simulink model "baseline_source"  (R2025a)
settings: Solver=daessc  StartTime=0.0  StopTime=25  MaxStep=5e-6  RelTol=1e-3
model workspace (MAT data in the model file):
  FocDiscrTime = 8.33333333333e-05
  Is_max = 420
  Ld = 0.00031
  Lq = 0.000305
  PolePairs = 11
  Psi = 0.1024
  Rs = 0.02
  VDC = 440
  compensate_dt = 0
  compensate_pwm = 0
  deltaLd = 0
  deltaLq = 0
  deltaPsi = 0
  deltaRs = 0
  mFW = 0.95
  mMaxCurrent = 0.99
  mMaxPWM = 0.99
  piBandwidth = 6000
libraries: fl_lib x18, nesl_utility x15, eeGeneralControl x9, mcbeeMathTransformLib x7, simulink x7, slpidlib x5, spsMeanLib x4, ee_lib x1, simulink_extras x1
(part 2 of 2)

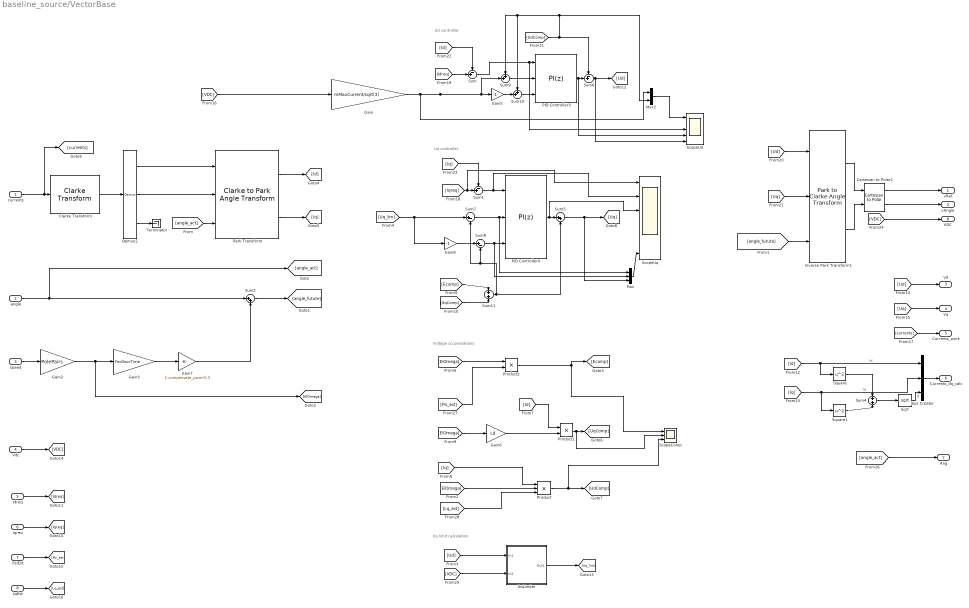
== system baseline_source/VectorBase ==
  note: Uq limit calculation
  note: Voltage co,pensations
  note: Ud controller
  note: Uq controller
  currents : Inport
  angle : Inport  Port=2
  speed : Inport  Port=3
  Vdc : Inport  Port=4
  Idreq : Inport  Port=5
  Iqreq : Inport  Port=6
  PsiEst : Inport  Port=7
  LqEst : Inport  Port=8
  Bus Creator : BusCreator  Inputs=3
  Cartesian to Polar1 : simulink_extras/Transformations/Cartesian to Polar
  Clarke Transform : mcbeeMathTransformLib/Clarke Transform  VariantControl=Variant2  PowerInvariant=off  UseWithEmbedded=on  PhaseInput=Three inputs
      settings: LibrarySourceBlock=mcbcontrolslib/Clarke Transform
  Demux2 : Demux  Outputs=3
  Gain : Gain  Gain=mMaxCurrent/sqrt(3)
  Gain2 : Gain  Gain=PolePairs
  Gain3 : Gain  Gain=FocDiscrTime
  Gain5 : Gain  Gain=-1
  Gain6 : Gain  Gain=Ld
  Gain7 : Gain  Gain=1-compensate_pwm*0.5
  Gain8 : Gain  Gain=-1
  Inverse Park Transform1 : mcbeeMathTransformLib/Park to Clarke Angle Transform  AxisAlignment=D-axis  UseWithEmbedded=on  PhaseInput=Two inputs  ThetaInput=Electrical position  AngleInput=Radians  N_points=1024
      settings: LibrarySourceBlock=mcbcontrolslib/Inverse Park Transform
  Mux : Mux  Inputs=3
  Mux2 : Mux  Inputs=2
  PID Controller3 : slpidlib/PID Controller  Controller=PI  Form=Parallel  TimeDomain=Discrete-time  UseExternalTs=off  SampleTime=FocDiscrTime  IntegratorMethod=Forward Euler  FilterMethod=Forward Euler  ControllerParametersSource=internal  P=piBandwidth*Ld  I=piBandwidth*Rs  UseKiTs=off  D=0  UseExternalDerivativeSource=off  N=100  UseFilter=on  TunerSelectOption=Transfer Function Based (PID Tuner App)  InitialConditionSource=internal  InitialConditionForIntegrator=0  InitialConditionForFilter=0  DifferentiatorICPrevScaledInput=0  ExternalReset=none  TrackingMode=off  Kt=1  LimitOutput=on  SatLimitsSource=external  UpperSaturationLimit=0  LowerSaturationLimit=0  LinearizeAsGain=on  AntiWindupMode=clamping  Kb=1  LimitIntegrator=off  UpperIntegratorSaturationLimit=inf  LowerIntegratorSaturationLimit=-inf  POutMin=[]  POutMax=[]  IOutMin=[]  IOutMax=[]  DOutMin=[]  DOutMax=[]  NOutMin=[]  NOutMax=[]  SumOutMin=[]  SumOutMax=[]  SaturationOutMin=[]  SaturationOutMax=[]  PParamMin=[]  PParamMax=[]  IParamMin=[]  IParamMax=[]  DParamMin=[]  DParamMax=[]  NParamMin=[]  NParamMax=[]  KbParamMin=[]  KbParamMax=[]  KtParamMin=[]  KtParamMax=[]  KbOutMin=[]  KbOutMax=[]  KtOutMin=[]  KtOutMax=[]  IntegratorOutMin=[]  IntegratorOutMax=[]  FilterOutMin=[]  FilterOutMax=[]  SumI1OutMin=[]  SumI1OutMax=[]  SumI2OutMin=[]  SumI2OutMax=[]  SumI3OutMin=[]  SumI3OutMax=[]  SumI4OutMin=[]  SumI4OutMax=[]  SumDOutMin=[]  SumDOutMax=[]  DifferentiatorOutMin=[]  DifferentiatorOutMax=[]  FilterDiffOutCoefMin=[]  FilterDiffOutCoefMax=[]  ReciprocalOutMin=[]  ReciprocalOutMax=[]  SumDenOutMin=[]  SumDenOutMax=[]  SumNumOutMin=[]  SumNumOutMax=[]  DivideOutMin=[]  DivideOutMax=[]  UdiffTsProdOutMin=[]  UdiffTsProdOutMax=[]  NTsProdOutMin=[]  NTsProdOutMax=[]  UintegralTsProdOutMin=[]  UintegralTsProdOutMax=[]  UngainTsProdOutMin=[]  UngainTsProdOutMax=[]  ClampingZeroOutDataTypeStr=Inherit: Inherit via back propagation  ClampingZeroOutMin=[]  ClampingZeroOutMax=[]  FilterDenConstantOutDataTypeStr=Inherit: Inherit via back propagation  FilterDenConstantOutMin=[]  FilterDenConstantOutMax=[]  PCopyOutDataTypeStr=Inherit: Inherit via back propagation  PCopyOutMin=[]  PCopyOutMax=[]  NCopyOutDataTypeStr=Inherit: Inherit via back propagation  NCopyOutMin=[]  NCopyOutMax=[]  IntegratorContinuousStateAttributes=''  IntegratorStateMustResolveToSignalObject=off  IntegratorRTWStateStorageClass=Auto  FilterContinuousStateAttributes=''  FilterStateMustResolveToSignalObject=off  FilterRTWStateStorageClass=Auto  ParallelPVariant=InternalParameters  IdealPVariant=Disabled  IVariant=InternalParameters  DVariant=Disabled  IntegratorVariant=Discrete  SatVariant=External  AWVariant=DiscClampingParallel  PCopyVariant=Disabled  TRVariant=Disabled  FdbkBlocksVariant=Forward  IdealPFdbkVariant=Disabled  SatFdbkVariant=Disabled  DerivativeFilterVariant=Disabled  NVariant=Disabled  NCopyVariant=Disabled_SignalSpec  FilterICVariant=Disabled  IntegratorICVariant=InternalICs  ExternalResetVariant=Disabled  TRSumVariant=Passthrough  SumFdbkVariant=Disabled  SumVariant=Sum_PI  TsampFilterVariant=InternalTs  TsampNgainVariant=Passthrough  TsampIntegralVariant=Disabled_SignalSpec  ExternalSaturationOutDataTypeStr=Inherit: Same as second input  DerivativeSourceVariant=Disabled  PreIntVariant=InternalPreInt
  PID Controller4 : slpidlib/PID Controller  Controller=PI  Form=Parallel  TimeDomain=Discrete-time  UseExternalTs=off  SampleTime=FocDiscrTime  IntegratorMethod=Forward Euler  FilterMethod=Forward Euler  ControllerParametersSource=internal  P=piBandwidth*Lq  I=piBandwidth*Rs  UseKiTs=off  D=0  UseExternalDerivativeSource=off  N=100  UseFilter=on  TunerSelectOption=Transfer Function Based (PID Tuner App)  InitialConditionSource=internal  InitialConditionForIntegrator=0  InitialConditionForFilter=0  DifferentiatorICPrevScaledInput=0  ExternalReset=none  TrackingMode=off  Kt=1  LimitOutput=on  SatLimitsSource=external  UpperSaturationLimit=24  LowerSaturationLimit=-15  LinearizeAsGain=on  AntiWindupMode=clamping  Kb=1  LimitIntegrator=off  UpperIntegratorSaturationLimit=inf  LowerIntegratorSaturationLimit=-inf  POutMin=[]  POutMax=[]  IOutMin=[]  IOutMax=[]  DOutMin=[]  DOutMax=[]  NOutMin=[]  NOutMax=[]  SumOutMin=[]  SumOutMax=[]  SaturationOutMin=[]  SaturationOutMax=[]  PParamMin=[]  PParamMax=[]  IParamMin=[]  IParamMax=[]  DParamMin=[]  DParamMax=[]  NParamMin=[]  NParamMax=[]  KbParamMin=[]  KbParamMax=[]  KtParamMin=[]  KtParamMax=[]  KbOutMin=[]  KbOutMax=[]  KtOutMin=[]  KtOutMax=[]  IntegratorOutMin=[]  IntegratorOutMax=[]  FilterOutMin=[]  FilterOutMax=[]  SumI1OutMin=[]  SumI1OutMax=[]  SumI2OutMin=[]  SumI2OutMax=[]  SumI3OutMin=[]  SumI3OutMax=[]  SumI4OutMin=[]  SumI4OutMax=[]  SumDOutMin=[]  SumDOutMax=[]  DifferentiatorOutMin=[]  DifferentiatorOutMax=[]  FilterDiffOutCoefMin=[]  FilterDiffOutCoefMax=[]  ReciprocalOutMin=[]  ReciprocalOutMax=[]  SumDenOutMin=[]  SumDenOutMax=[]  SumNumOutMin=[]  SumNumOutMax=[]  DivideOutMin=[]  DivideOutMax=[]  UdiffTsProdOutMin=[]  UdiffTsProdOutMax=[]  NTsProdOutMin=[]  NTsProdOutMax=[]  UintegralTsProdOutMin=[]  UintegralTsProdOutMax=[]  UngainTsProdOutMin=[]  UngainTsProdOutMax=[]  ClampingZeroOutDataTypeStr=Inherit: Inherit via back propagation  ClampingZeroOutMin=[]  ClampingZeroOutMax=[]  FilterDenConstantOutDataTypeStr=Inherit: Inherit via back propagation  FilterDenConstantOutMin=[]  FilterDenConstantOutMax=[]  PCopyOutDataTypeStr=Inherit: Inherit via back propagation  PCopyOutMin=[]  PCopyOutMax=[]  NCopyOutDataTypeStr=Inherit: Inherit via back propagation  NCopyOutMin=[]  NCopyOutMax=[]  IntegratorContinuousStateAttributes=''  IntegratorStateMustResolveToSignalObject=off  IntegratorRTWStateStorageClass=Auto  FilterContinuousStateAttributes=''  FilterStateMustResolveToSignalObject=off  FilterRTWStateStorageClass=Auto  ParallelPVariant=InternalParameters  IdealPVariant=Disabled  IVariant=InternalParameters  DVariant=Disabled  IntegratorVariant=Discrete  SatVariant=External  AWVariant=DiscClampingParallel  PCopyVariant=Disabled  TRVariant=Disabled  FdbkBlocksVariant=Forward  IdealPFdbkVariant=Disabled  SatFdbkVariant=Disabled  DerivativeFilterVariant=Disabled  NVariant=Disabled  NCopyVariant=Disabled_SignalSpec  FilterICVariant=Disabled  IntegratorICVariant=InternalICs  ExternalResetVariant=Disabled  TRSumVariant=Passthrough  SumFdbkVariant=Disabled  SumVariant=Sum_PI  TsampFilterVariant=InternalTs  TsampNgainVariant=Passthrough  TsampIntegralVariant=Disabled_SignalSpec  ExternalSaturationOutDataTypeStr=Inherit: Same as second input  DerivativeSourceVariant=Disabled  PreIntVariant=InternalPreInt
  Park Transform : mcbeeMathTransformLib/Clarke to Park Angle Transform  AxisAlignment=D-axis  UseWithEmbedded=on  PhaseInput=Two inputs  ThetaInput=Electrical position  AngleInput=Radians  N_points=1024
      settings: LibrarySourceBlock=mcbcontrolslib/Park Transform
  Product : Product  Inputs=3
  Product1 : Product
  Product2 : Product
  ScopeComp : Scope  NumInputPorts=3
      settings: ActiveDisplayYMinimum=-1056.5928598583193  ActiveDisplayYMaximum=1041.0472066509114
  ScopeUd : Scope  NumInputPorts=5
      settings: ActiveDisplayYMinimum=-149.14017921738167  ActiveDisplayYMaximum=299.51459067540895  DataLoggingVariableName=ScopeData6
  ScopeUq : Scope  NumInputPorts=6
      settings: ActiveDisplayYMinimum=-99.749999605061  ActiveDisplayYMaximum=477.74999644554919  DataLoggingVariableName=ScopeData4
  Sqrt : Sqrt
  Square : Math  Operator=square
  Square1 : Math  Operator=square
  Sum : Sum  Inputs=-+|
  Sum1 : Sum  Inputs=-+|
  Sum10 : Sum  Inputs=++|
  Sum11 : Sum
  Sum2 : Sum  Inputs=|++
  Sum4 : Sum
  Sum5 : Sum  Inputs=|++
  Sum6 : Sum  Inputs=-+|
  Sum7 : Sum  Inputs=|+-
  Sum8 : Sum  Inputs=|+-
  Sum9 : Sum  Inputs=++|
  Terminator : Terminator
  UqLimiter : Subsystem
  vRef : Outport
  vAngle : Outport  Port=2
  Vd : Outport  Port=3
  Vq : Outport  Port=4
  Currents_work : Outport  Port=5
  Currents_dq_calc : Outport  Port=6
  Ang : Outport  Port=7
  VDC : Outport  Port=8
  wires:
  Sum5/1 -> Mux/3, [Uq]
  Mux/1 -> ScopeUq/6
  Sqrt/1 -> Bus Creator/3  "Is"
  Sum4/1 -> Sqrt/1
  Square1/1 -> Sum4/2
  Square/1 -> Sum4/1
  [VDC] -> VDC/1
  Cartesian to Polar1/1 -> vRef/1
  Cartesian to Polar1/2 -> vAngle/1
  [angle_act] -> Ang/1
  Gain7/1 -> Sum2/2
  Gain5/1 -> Sum10/2
  Gain/1 -> Mux2/1, Sum9/2, Gain5/1
  [VDC] -> Gain/1
  Vdc/1 -> [VDC]
  [Iq] -> Sum1/1
  [Id] -> Sum/1
  [Uq] -> Inverse Park Transform1/2
  [Ud] -> Inverse Park Transform1/1
  Iqreq/1 -> [Iqreq]
  Idreq/1 -> [Idreq]
  [currents] -> Currents_work/1
  Sum7/1 -> PID Controller4/2, Mux/1
  [Uq] -> Vq/1
  [Ud] -> Vd/1
  [Iq] -> Bus Creator/2, Square1/1  "Iq"
  [Id] -> Bus Creator/1, Square/1  "Id"
  Product/1 -> [UdComp], ScopeComp/3
  Product1/1 -> [UqComp], ScopeComp/2
  [ElOmega] -> Gain6/1
  [Iq] -> Product/1
  [Id] -> Product1/1
  [ElOmega] -> Product2/1
  Product2/1 -> [Ecomp], ScopeComp/1
  Gain3/1 -> Gain7/1
  Gain2/1 -> Gain3/1, [ElOmega]
  UqLimiter/1(Out1) -> [Uq_lim]
  [VDC] -> UqLimiter/2(In2)
  [Ud] -> UqLimiter/1(In1)
  [UdComp] -> Sum10/1, Sum9/1, Mux2/2, Sum6/1
  Gain6/1 -> Product1/2
  [ElOmega] -> Product/2
  [angle_futute] -> Inverse Park Transform1/3
  [angle_act] -> Park Transform/3
  Bus Creator/1 -> Currents_dq_calc/1
  PID Controller3/1 -> ScopeUd/4, Sum6/2
  Inverse Park Transform1/2 -> Cartesian to Polar1/2
  Inverse Park Transform1/1 -> Cartesian to Polar1/1
  Sum8/1 -> PID Controller4/3, Mux/2
  Sum1/1 -> PID Controller4/1, ScopeUq/2
  PID Controller4/1 -> Sum5/1, ScopeUq/3
  Park Transform/1 -> [Id]
  Demux2/2 -> Park Transform/2
  Sum/1 -> ScopeUd/3, PID Controller3/1
  Clarke Transform/1 -> Demux2/1
  [Iqreq] -> Sum1/2, ScopeUq/1
  Demux2/3 -> Terminator/1
  Park Transform/2 -> [Iq]
  Demux2/1 -> Park Transform/1
  currents/1 -> Clarke Transform/1, [currents]
  Sum2/1 -> [angle_futute]
  angle/1 -> Sum2/1, [angle_act]
  speed/1 -> Gain2/1
  Sum6/1 -> ScopeUd/5, [Ud]
  [Idreq] -> Sum/2
  [Uq_lim] -> Sum7/1, Gain8/1
  [Psi_est] -> Product2/2
  PsiEst/1 -> [Psi_est]
  Mux2/1 -> ScopeUd/1
  Gain8/1 -> Sum8/1
  [UqComp] -> Sum11/2
  [Ecomp] -> Sum11/1
  Sum11/1 -> Sum5/2, Sum7/2, Sum8/2
  LqEst/1 -> [Lq_est]
  [Lq_est] -> Product/3
  Sum9/1 -> PID Controller3/2
  Sum10/1 -> PID Controller3/3

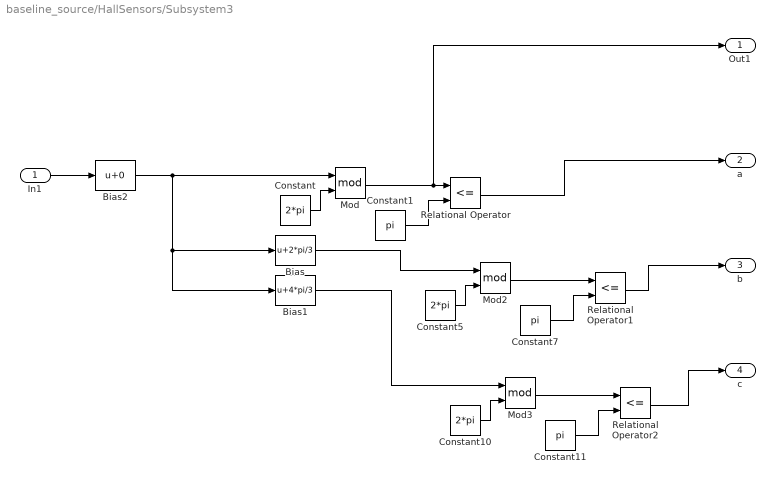
== system baseline_source/HallSensors/Subsystem3 ==
  In1 : Inport
  Bias : Bias  Bias=2*pi/3  SaturateOnIntegerOverflow=off
  Bias1 : Bias  Bias=4*pi/3  SaturateOnIntegerOverflow=off
  Bias2 : Bias  SaturateOnIntegerOverflow=off
  Constant : Constant  Value=2*pi
  Constant1 : Constant  Value=pi
  Constant10 : Constant  Value=2*pi
  Constant11 : Constant  Value=pi
  Constant5 : Constant  Value=2*pi
  Constant7 : Constant  Value=pi
  Mod : Math  Operator=mod
  Mod2 : Math  Operator=mod
  Mod3 : Math  Operator=mod
  Relational Operator : RelationalOperator  Operator=<=  OutDataTypeStr=boolean  RndMeth=Simplest  InputSameDT=off
  Relational Operator1 : RelationalOperator  Operator=<=  OutDataTypeStr=boolean  RndMeth=Simplest  InputSameDT=off
  Relational Operator2 : RelationalOperator  Operator=<=  OutDataTypeStr=boolean  RndMeth=Simplest  InputSameDT=off
  Out1 : Outport
  "a " : Outport  Port=2
  b : Outport  Port=3
  c : Outport  Port=4
  wires:
  Bias/1 -> Mod2/1
  Constant5/1 -> Mod2/2
  Relational Operator1/1 -> b/1
  Relational Operator2/1 -> c/1
  Constant7/1 -> Relational Operator1/2
  Mod/1 -> Out1/1, Relational Operator/1
  Bias1/1 -> Mod3/1
  Mod2/1 -> Relational Operator1/1
  Constant11/1 -> Relational Operator2/2
  Constant10/1 -> Mod3/2
  Constant/1 -> Mod/2
  Constant1/1 -> Relational Operator/2
  Relational Operator/1 -> "a "/1
  Mod3/1 -> Relational Operator2/1
  In1/1 -> Bias2/1
  Bias2/1 -> Bias1/1, Bias/1, Mod/1

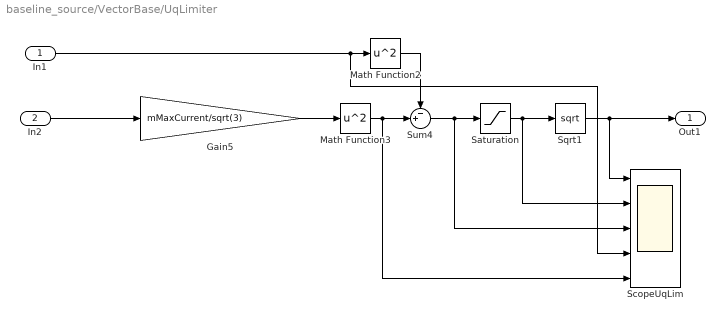
== system baseline_source/VectorBase/UqLimiter ==
  In1 : Inport
  In2 : Inport  Port=2
  Gain5 : Gain  Gain=mMaxCurrent/sqrt(3)
  Math Function2 : Math  Operator=square
  Math Function3 : Math  Operator=square
  Saturation : Saturate  UpperLimit=inf  LowerLimit=0.001
  ScopeUqLim : Scope  NumInputPorts=5
      settings: ActiveDisplayYMinimum=149.70176366248859  ActiveDisplayYMaximum=275.51811800976793  DataLoggingVariableName=ScopeData5
  Sqrt1 : Sqrt
  Sum4 : Sum  Inputs=-+|
  Out1 : Outport
  wires:
  In1/1 -> Math Function2/1, ScopeUqLim/4
  Sqrt1/1 -> Out1/1, ScopeUqLim/1
  Sum4/1 -> Saturation/1, ScopeUqLim/3
  Math Function2/1 -> Sum4/1
  In2/1 -> Gain5/1
  Gain5/1 -> Math Function3/1
  Math Function3/1 -> Sum4/2, ScopeUqLim/5
  Saturation/1 -> Sqrt1/1, ScopeUqLim/2

== matlab function baseline_source/MATLAB Function ==
  data: u input; y output
function y = fcn(u)
%#codegen

if u >= 0 && u < 0.1
    y = 0.1;
elseif u < 0 && u > -0.1
    y = -0.1;
else 
    y = u;
end

== matlab function baseline_source/sat_signed1 ==
  data: u input; y output
function y = fcn(u)
%#codegen
s = max(abs(u), 40);      % floor модуля

if u >= 0, y = s; else, y = -s; end

== matlab function baseline_source/sat_signed2 ==
  data: u input; y output
function y = fcn(u)
%#codegen
s = max(abs(u), 40);      % floor модуля

if u >= 0, y = s; else, y = -s; end

== matlab function baseline_source/sat_signed3 ==
  data: u input; y output
function y = fcn(u)
%#codegen
s = max(abs(u), 0.1);      % floor модуля

if u >= 0, y = s; else, y = -s; end

== matlab function baseline_source/sat_signed4 ==
  data: u input; y output
function y = fcn(u)
%#codegen
s = max(abs(u), 0.1);      % floor модуля

if u >= 0, y = s; else, y = -s; end

== matlab function baseline_source/sat_signed5 ==
  data: u input; y output
function y = fcn(u)
%#codegen
s = max(abs(u), 0.1);      % floor модуля

if u >= 0, y = s; else, y = -s; end

== matlab function baseline_source/Min_smooth_ab ==
  data: a input; y output; b input
function y = fcn(a,b)
%#codegen
delta = 10; %A
y = 0.5 * ((a+b) - sqrt((a-b)^2 + delta^2));

== matlab function baseline_source/HallSensors/MATLAB Function ==
  data: a input; ag output; b input; c input; s output
function [ag,s]= fcn(a,b,c)

dt = 1/20000;
persistent Speed;
if isempty(Speed)
    Speed = 0;
end

persistent Speed_flt;
if isempty(Speed_flt)
    Speed_flt = 0;
end


persistent cnt
if isempty(cnt)
    cnt = 0;
end

persistent com_cnt
if isempty(com_cnt)
    com_cnt = 0;
end


y = a + b * 2 + c *4;
if y == 3
    ar = pi/6;
elseif y == 1
    ar = 3*pi/6;
elseif y == 5
    ar = 5*pi/6;
elseif y == 4
    ar = 7*pi/6;
elseif y == 6
    ar = 9*pi/6;
elseif y == 2
    ar = 11*pi/6;
else 
    ar = 0;
end

ar = ar-pi/6;

persistent Angle;
if isempty(Angle)
    Angle = ar;
end

if ar ~= Angle
    f = ar - Angle;
    if f<0 
        f = f + 2*pi;
    end
    Speed_new = f/dt / (cnt+1);
    if abs(Speed_new - Speed) <  max(abs(Speed*0.5),500)
        Speed = Speed_new;
    end
    cnt = 0; 
else 
    cnt = cnt + 1;
end

%if Speed > 10000
%    Speed = 0;
%end



alfa = 0.0125;

Speed_flt = Speed_flt + alfa * (Speed - Speed_flt);

Angle = ar;







if Speed_flt < 500
    ag = ar;
else 
    ag = ar + Speed_flt*dt*(cnt +1);
end

while ag > 2*pi
    ag = ag - 2*pi;
end

s = Speed_flt;
end

== matlab function baseline_source/SVPWM1 ==
  data: vRef input; vAngle input; VDC input; Currents input; Tat output; Tbt output; Tct output; vRefwork output; compensate_pwm parameter; FocDiscrTime parameter; compensate_dt parameter; overModulation output; viol output; mMaxPWM parameter
function [Tat, Tbt, Tct,vRefwork, overModulation,viol] = fcn(vRef,vAngle, VDC, Currents, compensate_pwm, FocDiscrTime, compensate_dt, mMaxPWM)
% Векторная ШИМ с экстраполяцией скважности и компенсацией мёртвого времени.
% Исправления относительно исходной версии:
%   1) Ветка удержания выдаёт последние ОГРАНИЧЕННЫЕ выходы (Tat_out...),
%      а не сырое Ta_old. Ta_old по-прежнему сырое - для экстраполятора.
%   2) vOtn ограничен с двух сторон через min/max, VDC защищён снизу.
%      min/max игнорируют NaN, поэтому NaN не проходит клампы.
%   3) Ранний выход при нечисловых входах (NaN/Inf) - удержание выхода.
%   4) Компенсация мёртвого времени перенесена ДО финальных клампов
%      и применяется только в активном полутакте (без двойного учёта).
%   5) Клампы выходов - последняя операция, через min/max.
 overModulation = 0;
 viol = 0;
% --- параметры ---
timeStamp=FocDiscrTime;
deadTime        = 0.0;          % мёртвое время, мкс

VDC_min         = 0.1;           % нижняя защита напряжения ЗПТ, В
dutyMax         = 0.995;
dutyMin         = 0.005;

dead_time = deadTime/(timeStamp*1e6);

% --- persistent-состояния ---
persistent Ta_old Tb_old Tc_old;              % сырые скважности (для экстраполятора)
if isempty(Ta_old)
    Ta_old = 0.5;  Tb_old = 0.5;  Tc_old = 0.5;
end
 
persistent Tat_out Tbt_out Tct_out;           % последние выданные (ограниченные) выходы
if isempty(Tat_out)
    Tat_out = 0.5; Tbt_out = 0.5; Tct_out = 0.5;
end
 
persistent interruptCnt
if isempty(interruptCnt)
    interruptCnt = true;
end


vRefwork = vRef;

% --- защита от нечисловых входов: удерживаем последний корректный выход ---
if ~isfinite(vRef) || ~isfinite(vAngle) || ~isfinite(VDC)
    Tat = Tat_out;  Tbt = Tbt_out;  Tct = Tct_out;
    interruptCnt = ~interruptCnt;
    return;
end




if (interruptCnt)
    if (vAngle < 0)
        a = vAngle + 2*pi;
    elseif vAngle > 2*pi
        a = vAngle - 2*pi;
    else
        a=vAngle;
    end

    % относительная амплитуда, двусторонний кламп (min/max отсекают и NaN)
    vOtn = sqrt(3)*vRef / max(VDC, VDC_min);
    vOtn = min(max(vOtn, 0), mMaxPWM);


    if a>=0 && a<pi/3 
        n=1;
    elseif  a>=pi/3 && a<2*pi/3 
        n=2;
    elseif  a>=2*pi/3 && a<pi 
        n=3;
    elseif  a>=pi && a<4*pi/3 
        n=4;
    elseif  a>=4*pi/3 && a<5*pi/3 
        n=5;
    else 
        n=6;

    end

    a_cor=a-(n-1)*pi/3;

    T1 = vOtn * sin(pi/3 - a_cor);
    T2 = vOtn * sin(a_cor);
    T0=1-T1-T2;

    Ta=0; 
    Tb=0; 
    Tc=0;

    switch n
        case 1
            Ta = T1 + T2 + T0/2;
            Tb = T2 + T0/2;
            Tc = T0/2;
       
        case 2
            Ta = T1 + T0/2;
            Tb = T1 + T2 + T0/2;
            Tc = T0/2;       
        
        case 3
            Ta = T0/2;
            Tb = T1 + T2 + T0/2;
            Tc = T2 + T0/2;    
        
        case 4
            Ta = T0/2;
            Tb = T1 + T0/2;
            Tc = T1 + T2 + T0/2;   
       
        case 5
            Ta = T2 + T0/2;
            Tb = T0/2;
            Tc = T1 + T2 + T0/2;     
        
        case 6
            Ta = T1 + T2 + T0/2;
            Tb = T0/2;
            Tc = T1 + T0/2;    
        
    end


% экстраполяция на полупериод вперёд (по сырым значениям - так задумано)
    if compensate_pwm == 1
        Tat = 2*Ta - Ta_old;
        Tbt = 2*Tb - Tb_old;
        Tct = 2*Tc - Tc_old;
    else
        Tat = Ta;
        Tbt = Tb;
        Tct = Tc;
    end

% компенсация мёртвого времени - ДО клампов, только в активном полутакте
    if compensate_dt == 1
        if Currents(1) > 0
            Tat = Tat - dead_time/2;
        else
            Tat = Tat + dead_time/2;
        end
        if Currents(2) > 0
            Tbt = Tbt - dead_time/2;
        else
            Tbt = Tbt + dead_time/2;
        end
        if -(Currents(1)+Currents(2)) > 0
            Tct = Tct - dead_time/2;
        else
            Tct = Tct + dead_time/2;
        end
    end
overModulation = 0;
    viol = max(0, Tat - dutyMax) + max(0, dutyMin - Tat) ...
     + max(0, Tbt - dutyMax) + max(0, dutyMin - Tbt) ...
     + max(0, Tct - dutyMax) + max(0, dutyMin - Tct);
overModulation = double(viol > 0);

% финальные клампы - последняя операция (min/max: NaN не проходит)
    Tat = min(max(Tat, dutyMin), dutyMax);
    Tbt = min(max(Tbt, dutyMin), dutyMax);
    Tct = min(max(Tct, dutyMin), dutyMax);
 
    % запоминаем состояния:
    Ta_old  = Ta;   Tb_old  = Tb;   Tc_old  = Tc;    % сырые - для экстраполятора
    Tat_out = Tat;  Tbt_out = Tbt;  Tct_out = Tct;   % ограниченные - для удержания



    else
    % ================= полутакт удержания =================
    % выдаём ровно то, что реально было на выходе в активном полутакте
    Tat = Tat_out;
    Tbt = Tbt_out;
    Tct = Tct_out;
   
    viol = max(0, Tat - dutyMax) + max(0, dutyMin - Tat) ...
     + max(0, Tbt - dutyMax) + max(0, dutyMin - Tbt) ...
     + max(0, Tct - dutyMax) + max(0, dutyMin - Tct);
overModulation = double(viol > 0);
end
 
interruptCnt = ~interruptCnt;
end
